simulink model "acf_rl_native"  (R2026b)
settings: Solver=ode4  StopTime=inf  FixedStep=3.3333333333333333e-06
InitFcn:
  | acf_select_actuator(bdroot);
model workspace (MAT data in the model file):
  acfControlVersion = 'force-observer-v1'
  acfImplementation = 'simple'
  acfLayoutVersion = 1
  p : object (value not decoded)
  pCompliant : object (value not decoded)
  pNearContact : object (value not decoded)
  pNoSprings : object (value not decoded)
  pRecommended : object (value not decoded)
symbols that are objects in the model workspace (value not decoded): p
undefined symbols (not defined in the file or in its folder): DiscIntNeverNeededParam
libraries: sl_discontinuities x1
(part 2 of 3)

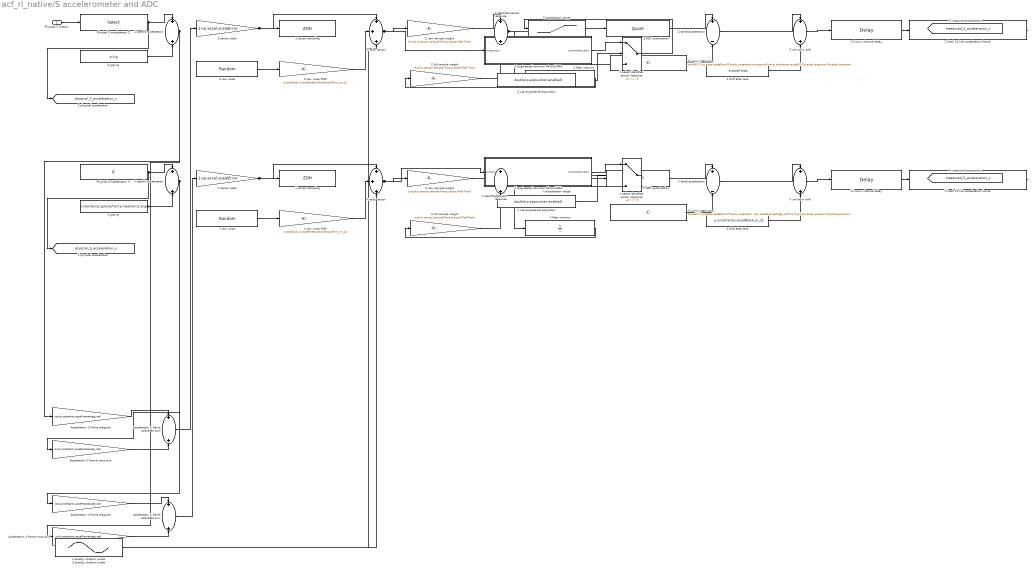
== system acf_rl_native/S accelerometer and ADC ==
  Physical S motion : Inport
  Acceleration X frame calibrated sum : Sum
  Acceleration X frame cross axis : Gain  Gain=-sin(p.uncertainty.accelFrameAngle_rad)
  Acceleration X frame diagonal : Gain  Gain=cos(p.uncertainty.accelFrameAngle_rad)
  Acceleration Z frame calibrated sum : Sum
  Acceleration Z frame cross axis : Gain  Gain=sin(p.uncertainty.accelFrameAngle_rad)
  Acceleration Z frame diagonal : Gain  Gain=cos(p.uncertainty.accelFrameAngle_rad)
  Physical S acceleration X : Constant  Value=0
  Physical S acceleration Z : Selector  InputPortWidth=3  IndexOptions=Index vector (dialog)  Indices=3  OutputSizes=1
  X ADC quantization : Quantizer  QuantizationInterval=1e-15
  X acceleration range : Saturate  UpperLimit=inf  LowerLimit=-inf
  X analog vibration probe : Sin  Amplitude=p.adcStudy.accelerationXAnalogToneAmplitude_m_s2  Frequency=2*pi*p.adcStudy.analogToneFrequency_Hz  Phase=p.adcStudy.analogTonePhase_rad  SampleTime=0
  X drift after tare : Constant  Value=p.uncertainty.accelBiasX_m_s2
  X engineered common AA and EMA : Subsystem
  X filter memory : UnitDelay  InitialCondition=(1+p.accel.scaleError)*(cos(p.uncertainty.accelFrameAngle_rad)*(p.mechanics.gravity*sin(p.mechanics.angle))-sin(p.uncertainty.accelFrameAngle_rad)*(p.d.g))  SampleTime=p.sensor.sampleTime
  X fresh 10 kHz acceleration frame : ZeroOrderHold  SampleTime=p.force.sampleTime
  X gravity : Constant  Value=p.mechanics.gravity*sin(p.mechanics.angle)
  X identified sensor response : Sum
  X known channel delay : TransportDelay  DelayTime=p.adcStudy.d.channels.acceleration.pipelineDelay_s  InitialOutput=p.uncertainty.accelBiasX_m_s2
  X known static tare : Constant  Value=round((((1+p.accel.scaleError)*(cos(p.uncertainty.accelFrameAngle_rad)*(p.mechanics.gravity*sin(p.mechanics.angle))-sin(p.uncertainty.accelFrameAngle_rad)*(p.d.g))))/p.accel.quantum)*p.accel.quantum
  X new sample weight : Gain  Gain=1-exp(-p.sensor.sampleTime/p.accel.filterTime)
  X noisy sensor : Sum  Inputs=+++
  X old sample weight : Gain  Gain=exp(-p.sensor.sampleTime/p.accel.filterTime)
  X raw noise : RandomNumber  Seed=p.sensor.seed+336  SampleTime=p.sensor.sampleTime
  X raw noise RMS : Gain  Gain=p.adcStudy.d.accelerationNoiseInputRms_m_s2
  X select identified sensor response : Switch  Threshold=.5  SaturateOnIntegerOverflow=off  InputSameDT=off
  X sensor sampling : ZeroOrderHold  SampleTime=p.sensor.sampleTime
  X sensor scale : Gain  Gain=1+p.accel.scaleError
  X specific acceleration : Sum
  X tared acceleration : Sum  Inputs=+-
  X unknown drift : Sum
  X use engineered acquisition : Constant  Value=double(p.acquisition.enabled)
  Z ADC quantization : Quantizer  QuantizationInterval=1e-15
  Z acceleration range : Saturate  UpperLimit=inf  LowerLimit=-inf
  Z analog vibration probe : Sin  Amplitude=p.adcStudy.accelerationZAnalogToneAmplitude_m_s2  Frequency=2*pi*p.adcStudy.analogToneFrequency_Hz  Phase=p.adcStudy.analogTonePhase_rad  SampleTime=0
  Z drift after tare : Constant  Value=p.accel.bias
  Z engineered common AA and EMA : Subsystem
  Z filter memory : UnitDelay  InitialCondition=(1+p.accel.scaleError)*(cos(p.uncertainty.accelFrameAngle_rad)*(p.d.g)+sin(p.uncertainty.accelFrameAngle_rad)*(p.mechanics.gravity*sin(p.mechanics.angle)))  SampleTime=p.sensor.sampleTime
  Z fresh 10 kHz acceleration frame : ZeroOrderHold  SampleTime=p.force.sampleTime
  Z gravity : Constant  Value=p.d.g
  Z identified sensor response : Sum
  Z known channel delay : TransportDelay  DelayTime=p.adcStudy.d.channels.acceleration.pipelineDelay_s  InitialOutput=p.accel.bias
  Z known static tare : Constant  Value=round((((1+p.accel.scaleError)*(cos(p.uncertainty.accelFrameAngle_rad)*(p.d.g)+sin(p.uncertainty.accelFrameAngle_rad)*(p.mechanics.gravity*sin(p.mechanics.angle)))))/p.accel.quantum)*p.accel.quantum
  Z new sample weight : Gain  Gain=1-exp(-p.sensor.sampleTime/p.accel.filterTime)
  Z noisy sensor : Sum  Inputs=+++
  Z old sample weight : Gain  Gain=exp(-p.sensor.sampleTime/p.accel.filterTime)
  Z raw noise : RandomNumber  Seed=p.sensor.seed+239  SampleTime=p.sensor.sampleTime
  Z raw noise RMS : Gain  Gain=p.adcStudy.d.accelerationNoiseInputRms_m_s2
  Z select identified sensor response : Switch  Threshold=.5  SaturateOnIntegerOverflow=off  InputSameDT=off
  Z sensor sampling : ZeroOrderHold  SampleTime=p.sensor.sampleTime
  Z sensor scale : Gain  Gain=1+p.accel.scaleError
  Z specific acceleration : Sum
  Z tared acceleration : Sum  Inputs=+-
  Z unknown drift : Sum
  Z use engineered acquisition : Constant  Value=double(p.acquisition.enabled)
  tag scope: measured_S_acceleration_x=global, measured_S_acceleration_z=global, physical_S_acceleration_x=global, physical_S_acceleration_z=global
  wires:
  Physical S motion/1 -> Physical S acceleration Z/1
  Physical S acceleration Z/1 -> [physical_S_acceleration_z], Z specific acceleration/1
  Z gravity/1 -> Z specific acceleration/2
  Z sensor scale/1 -> Z sensor sampling/1, Z noisy sensor/1
  Z raw noise/1 -> Z raw noise RMS/1
  Z raw noise RMS/1 -> Z noisy sensor/2
  Z noisy sensor/1 -> Z new sample weight/1, Z engineered common AA and EMA/1(analog input)
  Z new sample weight/1 -> Z identified sensor response/1
  Z identified sensor response/1 -> Z filter memory/1, Z select identified sensor response/3
  Z filter memory/1 -> Z old sample weight/1
  Z old sample weight/1 -> Z identified sensor response/2
  Z acceleration range/1 -> Z ADC quantization/1
  Z ADC quantization/1 -> Z tared acceleration/1
  Z known static tare/1 -> Z tared acceleration/2
  Z tared acceleration/1 -> Z unknown drift/1
  Z drift after tare/1 -> Z unknown drift/2
  Physical S acceleration X/1 -> [physical_S_acceleration_x], X specific acceleration/1
  X gravity/1 -> X specific acceleration/2
  X specific acceleration/1 -> Acceleration Z frame cross axis/1, Acceleration X frame diagonal/1
  X sensor scale/1 -> X sensor sampling/1, X noisy sensor/1
  X raw noise/1 -> X raw noise RMS/1
  X raw noise RMS/1 -> X noisy sensor/2
  X noisy sensor/1 -> X new sample weight/1, X engineered common AA and EMA/1(analog input)
  X new sample weight/1 -> X identified sensor response/1
  X identified sensor response/1 -> X filter memory/1, X select identified sensor response/3
  X filter memory/1 -> X old sample weight/1
  X old sample weight/1 -> X identified sensor response/2
  X acceleration range/1 -> X ADC quantization/1
  X ADC quantization/1 -> X tared acceleration/1
  X known static tare/1 -> X tared acceleration/2
  X tared acceleration/1 -> X unknown drift/1
  X drift after tare/1 -> X unknown drift/2
  Z use engineered acquisition/1 -> Z select identified sensor response/2
  Z select identified sensor response/1 -> Z acceleration range/1
  Z fresh 10 kHz acceleration frame/1 -> [measured_S_acceleration_z]
  X use engineered acquisition/1 -> X select identified sensor response/2
  X select identified sensor response/1 -> X acceleration range/1
  X fresh 10 kHz acceleration frame/1 -> [measured_S_acceleration_x]
  Z specific acceleration/1 -> Acceleration Z frame diagonal/1, Acceleration X frame cross axis/1
  Acceleration Z frame diagonal/1 -> Acceleration Z frame calibrated sum/1
  Acceleration Z frame cross axis/1 -> Acceleration Z frame calibrated sum/2
  Acceleration Z frame calibrated sum/1 -> Z sensor scale/1
  Acceleration X frame diagonal/1 -> Acceleration X frame calibrated sum/1
  Acceleration X frame cross axis/1 -> Acceleration X frame calibrated sum/2
  Acceleration X frame calibrated sum/1 -> X sensor scale/1
  Z analog vibration probe/1 -> Z noisy sensor/3
  Z engineered common AA and EMA/1(conditioned output) -> Z select identified sensor response/1
  Z unknown drift/1 -> Z known channel delay/1
  Z known channel delay/1 -> Z fresh 10 kHz acceleration frame/1
  X analog vibration probe/1 -> X noisy sensor/3
  X engineered common AA and EMA/1(conditioned output) -> X select identified sensor response/1
  X unknown drift/1 -> X known channel delay/1
  X known channel delay/1 -> X fresh 10 kHz acceleration frame/1

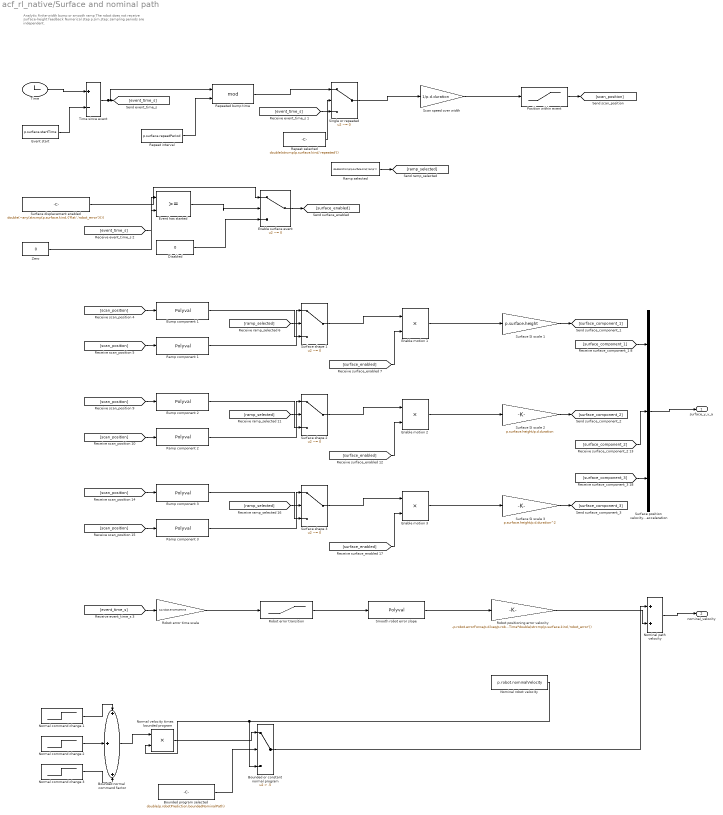
== system acf_rl_native/Surface and nominal path ==
  note: Analytic finite-width bump or smooth ramp
      | The robot does not receive surface-height feedback
      | Numerical step p.sim.step; sampling periods are independent.
  Bounded normal command factor : Sum  Inputs=+++
  Bounded or constant normal program : Switch  Criteria=u2 > Threshold  Threshold=.5  SaturateOnIntegerOverflow=off  InputSameDT=off
  Bounded program selected : Constant  Value=double(p.robotPrediction.boundedNominalPath)
  Bump component 1 : Polyval  Coefs=[-64 192 -192 64 0 0 0]
  Bump component 2 : Polyval  Coefs=[-384 960 -768 192 0 0]
  Bump component 3 : Polyval  Coefs=[-1920 3840 -2304 384 0]
  Disabled : Constant  Value=0
  Enable motion 1 : Product
  Enable motion 2 : Product
  Enable motion 3 : Product
  Enable surface event : Switch  Criteria=u2 ~= 0  SaturateOnIntegerOverflow=off  InputSameDT=off
  Event has started : RelationalOperator  OutDataTypeStr=boolean  RndMeth=Simplest  InputSameDT=off
  Event start : Constant  Value=p.surface.startTime
  Nominal path velocity : Sum
  Nominal robot velocity : Constant  Value=p.robot.nominalVelocity
  Normal command change 1 : Step  SampleTime=p.robot.sampleTime
  Normal command change 2 : Step  Time=2  FinalValue=-2  SampleTime=p.robot.sampleTime
  Normal command change 3 : Step  Time=3  SampleTime=p.robot.sampleTime
  Normal velocity times bounded program : Product
  Position within event : Saturate  UpperLimit=1  LowerLimit=0
  Ramp component 1 : Polyval  Coefs=[6 -15 10 0 0 0]
  Ramp component 2 : Polyval  Coefs=[30 -60 30 0 0]
  Ramp component 3 : Polyval  Coefs=[120 -180 60 0]
  Ramp selected : Constant  Value=double(strcmp(p.surface.kind,'ramp'))
  Repeat interval : Constant  Value=p.surface.repeatPeriod
  Repeat selected : Constant  Value=double(strcmp(p.surface.kind,'repeated'))
  Repeated bump time : Math  Operator=mod
  Robot error time scale : Gain  Gain=1/p.robot.errorRiseTime
  Robot error transition : Saturate  UpperLimit=1  LowerLimit=0
  Robot positioning error velocity : Gain  Gain=-p.robot.errorForce/p.d.keq/p.robot.errorRiseTime*double(strcmp(p.surface.kind,'robot_error'))
  Scan speed over width : Gain  Gain=1/p.d.duration
  Single or repeated : Switch  Criteria=u2 ~= 0  SaturateOnIntegerOverflow=off  InputSameDT=off
  Smooth robot error slope : Polyval  Coefs=[30 -60 30 0 0]
  Surface SI scale 1 : Gain  Gain=p.surface.height
  Surface SI scale 2 : Gain  Gain=p.surface.height/p.d.duration
  Surface SI scale 3 : Gain  Gain=p.surface.height/p.d.duration^2
  Surface displacement enabled : Constant  Value=double(~any(strcmp(p.surface.kind,{'flat','robot_error'})))
  Surface position velocity acceleration : Mux  Inputs=3
  Surface shape 1 : Switch  Criteria=u2 ~= 0  SaturateOnIntegerOverflow=off  InputSameDT=off
  Surface shape 2 : Switch  Criteria=u2 ~= 0  SaturateOnIntegerOverflow=off  InputSameDT=off
  Surface shape 3 : Switch  Criteria=u2 ~= 0  SaturateOnIntegerOverflow=off  InputSameDT=off
  Time : Clock
  Time since event : Sum  Inputs=+-
  Zero : Constant  Value=0
  surface_y_v_a : Outport
  nominal_velocity : Outport  Port=2
  wires:
  [scan_position] -> Bump component 1/1
  [scan_position] -> Bump component 2/1
  [scan_position] -> Bump component 3/1
  Surface shape 1/1 -> Enable motion 1/1
  [surface_enabled] -> Enable motion 1/2
  Surface shape 2/1 -> Enable motion 2/1
  [surface_enabled] -> Enable motion 2/2
  Surface shape 3/1 -> Enable motion 3/1
  [surface_enabled] -> Enable motion 3/2
  Surface displacement enabled/1 -> Enable surface event/1
  Event has started/1 -> Enable surface event/2
  Disabled/1 -> Enable surface event/3
  [event_time_s] -> Event has started/1
  Zero/1 -> Event has started/2
  Robot positioning error velocity/1 -> Nominal path velocity/2
  Scan speed over width/1 -> Position within event/1
  [scan_position] -> Ramp component 1/1
  [scan_position] -> Ramp component 2/1
  [scan_position] -> Ramp component 3/1
  Time since event/1 -> Repeated bump time/1, [event_time_s]
  Repeat interval/1 -> Repeated bump time/2
  [event_time_s] -> Robot error time scale/1
  Robot error time scale/1 -> Robot error transition/1
  Smooth robot error slope/1 -> Robot positioning error velocity/1
  Single or repeated/1 -> Scan speed over width/1
  Ramp selected/1 -> [ramp_selected]
  Position within event/1 -> [scan_position]
  Surface SI scale 1/1 -> [surface_component_1]
  Surface SI scale 2/1 -> [surface_component_2]
  Surface SI scale 3/1 -> [surface_component_3]
  Enable surface event/1 -> [surface_enabled]
  Repeated bump time/1 -> Single or repeated/1
  Repeat selected/1 -> Single or repeated/2
  [event_time_s] -> Single or repeated/3
  Robot error transition/1 -> Smooth robot error slope/1
  Enable motion 1/1 -> Surface SI scale 1/1
  Enable motion 2/1 -> Surface SI scale 2/1
  Enable motion 3/1 -> Surface SI scale 3/1
  [surface_component_1] -> Surface position velocity acceleration/1
  [surface_component_2] -> Surface position velocity acceleration/2
  [surface_component_3] -> Surface position velocity acceleration/3
  Ramp component 1/1 -> Surface shape 1/1
  [ramp_selected] -> Surface shape 1/2
  Bump component 1/1 -> Surface shape 1/3
  Ramp component 2/1 -> Surface shape 2/1
  [ramp_selected] -> Surface shape 2/2
  Bump component 2/1 -> Surface shape 2/3
  Ramp component 3/1 -> Surface shape 3/1
  [ramp_selected] -> Surface shape 3/2
  Bump component 3/1 -> Surface shape 3/3
  Time/1 -> Time since event/1
  Event start/1 -> Time since event/2
  Surface position velocity acceleration/1 -> surface_y_v_a/1
  Nominal path velocity/1 -> nominal_velocity/1
  Normal command change 1/1 -> Bounded normal command factor/1
  Normal command change 2/1 -> Bounded normal command factor/2
  Normal command change 3/1 -> Bounded normal command factor/3
  Bounded normal command factor/1 -> Normal velocity times bounded program/1
  Nominal robot velocity/1 -> Normal velocity times bounded program/2, Bounded or constant normal program/3
  Normal velocity times bounded program/1 -> Bounded or constant normal program/1
  Bounded program selected/1 -> Bounded or constant normal program/2
  Bounded or constant normal program/1 -> Nominal path velocity/1

== system acf_rl_native/Surface contact force ==
  Axial reaction : Inport
  Physical surface velocity : Inport  Port=2
  Axial reaction factor : Sum  Inputs=+-
  Friction times slope : Gain  Gain=p.contact.mu
  Lateral reaction : Product  Inputs=**/
  Lateral sign : Gain  Gain=-1
  Normal reaction : Product  Inputs=**/
  Normalizer : Math  Operator=sqrt
  Slope plus friction : Bias  Bias=p.contact.mu  SaturateOnIntegerOverflow=off
  Squared slope : Math  Operator=square
  Squared slope plus one : Bias  Bias=1  SaturateOnIntegerOverflow=off
  Surface slope : Gain  Gain=1/p.surface.scanSpeed
  Unity : Constant
  Velocity component : Selector  InputPortWidth=3  IndexOptions=Index vector (dialog)  Indices=2  OutputSizes=1
  tag scope: actual_contact_slope=global, lateral_contact_N=global, normal_contact_N=global
  wires:
  Physical surface velocity/1 -> Velocity component/1
  Velocity component/1 -> Surface slope/1
  Surface slope/1 -> Squared slope/1, Friction times slope/1, Slope plus friction/1, [actual_contact_slope]
  Squared slope/1 -> Squared slope plus one/1
  Squared slope plus one/1 -> Normalizer/1
  Unity/1 -> Axial reaction factor/1
  Friction times slope/1 -> Axial reaction factor/2
  Axial reaction/1 -> Normal reaction/1
  Normalizer/1 -> Normal reaction/2, Lateral reaction/3
  Axial reaction factor/1 -> Normal reaction/3
  Normal reaction/1 -> Lateral reaction/1, [normal_contact_N]
  Slope plus friction/1 -> Lateral reaction/2
  Lateral reaction/1 -> Lateral sign/1
  Lateral sign/1 -> [lateral_contact_N]

== system acf_rl_native/Actuator and RABS mechanics/Actuator ==
  Command : Inport
  Gap position velocity : Inport  Port=2
  Spring load : Inport  Port=3
  Ideal position : Subsystem  VariantControl=Ideal position
  Leadscrew : Subsystem  VariantControl=Leadscrew
  Voice coil : Subsystem  VariantControl=Voice coil
  Transmitted force : Outport
  Drive measurements : Outport  Port=2

== system acf_rl_native/Actuator and RABS mechanics/B to S spring and damper ==
  S position velocity : Inport
  B position velocity : Inport  Port=2
  Rigid reaction : Inport  Port=3
  Compliant or rigid link : VariantSource  VariantControlMode=label  LabelModeActiveChoice=Compliant  VariantControls={Compliant, Rigid}
  Damping : Gain  Gain=p.mechanics.c1
  Endpoint difference : Sum  Inputs=+-
  Preload : Constant  Value=p.d.q10
  Spring and damper force : Sum  Inputs=+++
  Spring displacement and relative velocity : Demux  Outputs=2
  Stiffness : Gain  Gain=p.mechanics.k1
  Spring force : Outport
  wires:
  Spring displacement and relative velocity/2 -> Damping/1
  S position velocity/1 -> Endpoint difference/1
  B position velocity/1 -> Endpoint difference/2
  Preload/1 -> Spring and damper force/1
  Stiffness/1 -> Spring and damper force/2
  Damping/1 -> Spring and damper force/3
  Endpoint difference/1 -> Spring displacement and relative velocity/1
  Spring displacement and relative velocity/1 -> Stiffness/1
  Spring and damper force/1 -> Compliant or rigid link/1
  Rigid reaction/1 -> Compliant or rigid link/2
  Compliant or rigid link/1 -> Spring force/1

== system acf_rl_native/Actuator and RABS mechanics/Mass A ==
  Actuator force : Inport
  Upper spring force : Inport  Port=2
  Gravity : Constant  Value=p.d.g
  Inverse mass : Gain  Gain=1/p.mechanics.mA
  Net applied force : Sum  Inputs=+-
  Newton acceleration : Sum  Inputs=+-
  Position : Integrator  InitialCondition=p.d.u0
  Position and velocity : Mux  Inputs=2
  Velocity : Integrator
  Position velocity : Outport
  Acceleration : Outport  Port=2
  wires:
  Net applied force/1 -> Inverse mass/1
  Actuator force/1 -> Net applied force/1
  Upper spring force/1 -> Net applied force/2
  Inverse mass/1 -> Newton acceleration/1
  Gravity/1 -> Newton acceleration/2
  Velocity/1 -> Position/1, [velocity_m_s]
  Position/1 -> Position and velocity/1
  [velocity_m_s] -> Position and velocity/2
  Newton acceleration/1 -> Velocity/1, Acceleration/1
  Position and velocity/1 -> Position velocity/1

== system acf_rl_native/Actuator and RABS mechanics/Mass B ==
  Lower spring force : Inport
  Actuator force : Inport  Port=2
  Gravity : Constant  Value=p.d.g
  Inverse mass : Gain  Gain=1/p.mechanics.mB
  Net applied force : Sum  Inputs=+-
  Newton acceleration : Sum  Inputs=+-
  Position : Integrator
  Position and velocity : Mux  Inputs=2
  Velocity : Integrator
  Position velocity : Outport
  Acceleration : Outport  Port=2
  wires:
  Net applied force/1 -> Inverse mass/1
  Lower spring force/1 -> Net applied force/1
  Actuator force/1 -> Net applied force/2
  Inverse mass/1 -> Newton acceleration/1
  Gravity/1 -> Newton acceleration/2
  Velocity/1 -> Position/1, [velocity_m_s]
  Position/1 -> Position and velocity/1
  [velocity_m_s] -> Position and velocity/2
  Newton acceleration/1 -> Velocity/1, Acceleration/1
  Position and velocity/1 -> Position velocity/1

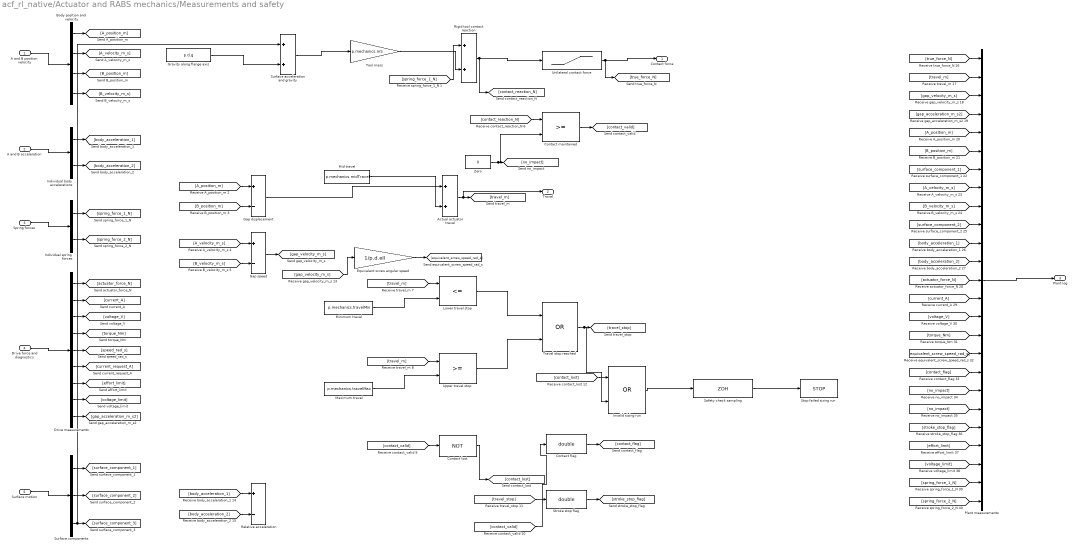
== system acf_rl_native/Actuator and RABS mechanics/Measurements and safety ==
  A and B position velocity : Inport
  A and B acceleration : Inport  Port=2
  Spring forces : Inport  Port=3
  Drive force and diagnostics : Inport  Port=4
  Surface motion : Inport  Port=5
  Actual actuator travel : Sum
  Body position and velocity : Demux
  Contact flag : DataTypeConversion  OutDataTypeStr=double  SaturateOnIntegerOverflow=off  RndMeth=Floor
  Contact lost : Logic  Operator=NOT  AllPortsSameDT=off  OutDataTypeStr=boolean
  Contact maintained : RelationalOperator  OutDataTypeStr=boolean  RndMeth=Simplest  InputSameDT=off
  Drive measurements : Demux  Outputs=9
  Equivalent screw angular speed : Gain  Gain=1/p.d.ell
  Gap displacement : Sum  Inputs=+-
  Gap speed : Sum  Inputs=+-
  Gravity along flange axis : Constant  Value=p.d.g
  Individual body accelerations : Demux  Outputs=2
  Individual spring forces : Demux  Outputs=2
  Invalid sizing run : Logic  Operator=OR  AllPortsSameDT=off  OutDataTypeStr=boolean
  Lower travel stop : RelationalOperator  Operator=<=  OutDataTypeStr=boolean  RndMeth=Simplest  InputSameDT=off
  Maximum travel : Constant  Value=p.mechanics.travelMax
  Mid travel : Constant  Value=p.mechanics.midTravel
  Minimum travel : Constant  Value=p.mechanics.travelMin
  Plant measurements : Mux  Inputs=25
  Relative acceleration : Sum  Inputs=+-
  Rigid tool contact reaction : Sum
  Safety check sampling : ZeroOrderHold  SampleTime=p.sim.step
  Stop failed sizing run : Stop
  Stroke stop flag : DataTypeConversion  OutDataTypeStr=double  SaturateOnIntegerOverflow=off  RndMeth=Floor
  Surface acceleration and gravity : Sum
  Surface components : Demux  Outputs=3
  Tool mass : Gain  Gain=p.mechanics.mS
  Travel stop reached : Logic  Operator=OR  AllPortsSameDT=off  OutDataTypeStr=boolean
  Unilateral contact force : Saturate  UpperLimit=inf  LowerLimit=0
  Upper travel stop : RelationalOperator  OutDataTypeStr=boolean  RndMeth=Simplest  InputSameDT=off
  Zero : Constant  Value=0
  Contact force : Outport
  Travel : Outport  Port=2
  Plant log : Outport  Port=3
  wires:
  Gap displacement/1 -> Actual actuator travel/1
  Mid travel/1 -> Actual actuator travel/2
  A and B position velocity/1 -> Body position and velocity/1
  [contact_valid] -> Contact flag/1
  [contact_valid] -> Contact lost/1
  [contact_reaction_N] -> Contact maintained/1
  Zero/1 -> Contact maintained/2, [no_impact]
  Drive force and diagnostics/1 -> Drive measurements/1
  [gap_velocity_m_s] -> Equivalent screw angular speed/1
  [A_position_m] -> Gap displacement/1
  [B_position_m] -> Gap displacement/2
  [A_velocity_m_s] -> Gap speed/1
  [B_velocity_m_s] -> Gap speed/2
  A and B acceleration/1 -> Individual body accelerations/1
  Spring forces/1 -> Individual spring forces/1
  [contact_lost] -> Invalid sizing run/1
  Travel stop reached/1 -> Invalid sizing run/2, [travel_stop]
  [travel_m] -> Lower travel stop/1
  Minimum travel/1 -> Lower travel stop/2
  [true_force_N] -> Plant measurements/1
  [travel_m] -> Plant measurements/2
  [gap_velocity_m_s] -> Plant measurements/3
  [gap_acceleration_m_s2] -> Plant measurements/4
  [A_position_m] -> Plant measurements/5
  [B_position_m] -> Plant measurements/6
  [surface_component_1] -> Plant measurements/7
  [A_velocity_m_s] -> Plant measurements/8
  [B_velocity_m_s] -> Plant measurements/9
  [surface_component_2] -> Plant measurements/10
  [body_acceleration_1] -> Plant measurements/11
  [body_acceleration_2] -> Plant measurements/12
  [actuator_force_N] -> Plant measurements/13
  [current_A] -> Plant measurements/14
  [voltage_V] -> Plant measurements/15
  [torque_Nm] -> Plant measurements/16
  [equivalent_screw_speed_rad_s] -> Plant measurements/17
  [contact_flag] -> Plant measurements/18
  [no_impact] -> Plant measurements/19
  [no_impact] -> Plant measurements/20
  [stroke_stop_flag] -> Plant measurements/21
  [effort_limit] -> Plant measurements/22
  [voltage_limit] -> Plant measurements/23
  [spring_force_1_N] -> Plant measurements/24
  [spring_force_2_N] -> Plant measurements/25
  [body_acceleration_1] -> Relative acceleration/1
  [body_acceleration_2] -> Relative acceleration/2
  [spring_force_1_N] -> Rigid tool contact reaction/1
  Tool mass/1 -> Rigid tool contact reaction/2
  Invalid sizing run/1 -> Safety check sampling/1
  Body position and velocity/1 -> [A_position_m]
  Body position and velocity/2 -> [A_velocity_m_s]
  Body position and velocity/3 -> [B_position_m]
  Body position and velocity/4 -> [B_velocity_m_s]
  Drive measurements/1 -> [actuator_force_N]
  Individual body accelerations/1 -> [body_acceleration_1]
  Individual body accelerations/2 -> [body_acceleration_2]
  Contact flag/1 -> [contact_flag]
  Contact lost/1 -> [contact_lost]
  Rigid tool contact reaction/1 -> [contact_reaction_N], Unilateral contact force/1
  Contact maintained/1 -> [contact_valid]
  Drive measurements/2 -> [current_A]
  Drive measurements/6 -> [current_request_A]
  Drive measurements/7 -> [effort_limit]
  Equivalent screw angular speed/1 -> [equivalent_screw_speed_rad_s]
  Drive measurements/9 -> [gap_acceleration_m_s2]
  Gap speed/1 -> [gap_velocity_m_s]
  Drive measurements/5 -> [speed_rad_s]
  Individual spring forces/1 -> [spring_force_1_N]
  Individual spring forces/2 -> [spring_force_2_N]
  Stroke stop flag/1 -> [stroke_stop_flag]
  Surface components/1 -> [surface_component_1]
  Surface components/2 -> [surface_component_2]
  Surface components/3 -> [surface_component_3], Surface acceleration and gravity/1
  Drive measurements/4 -> [torque_Nm]
  Actual actuator travel/1 -> [travel_m], Travel/1
  Unilateral contact force/1 -> [true_force_N], Contact force/1
  Drive measurements/3 -> [voltage_V]
  Drive measurements/8 -> [voltage_limit]
  Safety check sampling/1 -> Stop failed sizing run/1
  [travel_stop] -> Stroke stop flag/1
  Gravity along flange axis/1 -> Surface acceleration and gravity/2
  Surface motion/1 -> Surface components/1
  Surface acceleration and gravity/1 -> Tool mass/1
  Lower travel stop/1 -> Travel stop reached/1
  Upper travel stop/1 -> Travel stop reached/2
  [travel_m] -> Upper travel stop/1
  Maximum travel/1 -> Upper travel stop/2
  Plant measurements/1 -> Plant log/1

== system acf_rl_native/Actuator and RABS mechanics/R to A spring and damper ==
  A position velocity : Inport
  R position velocity : Inport  Port=2
  Rigid reaction : Inport  Port=3
  Compliant or rigid link : VariantSource  VariantControlMode=label  LabelModeActiveChoice=Rigid  VariantControls={Compliant, Rigid}
  Damping : Gain  Gain=p.mechanics.c2
  Endpoint difference : Sum  Inputs=+-
  Preload : Constant  Value=p.d.q20
  Spring and damper force : Sum  Inputs=+++
  Spring displacement and relative velocity : Demux  Outputs=2
  Stiffness : Gain  Gain=p.mechanics.k2
  Spring force : Outport
  wires:
  Spring displacement and relative velocity/2 -> Damping/1
  A position velocity/1 -> Endpoint difference/1
  R position velocity/1 -> Endpoint difference/2
  Preload/1 -> Spring and damper force/1
  Stiffness/1 -> Spring and damper force/2
  Damping/1 -> Spring and damper force/3
  Endpoint difference/1 -> Spring displacement and relative velocity/1
  Spring displacement and relative velocity/1 -> Stiffness/1
  Spring and damper force/1 -> Compliant or rigid link/1
  Rigid reaction/1 -> Compliant or rigid link/2
  Compliant or rigid link/1 -> Spring force/1

== system acf_rl_native/Contact force measurement/Contact force reconstruction ==
  raw_cell_error_N : Inport
  Cell error to deviation : Gain  Gain=-1
  Compensated axial reaction : Sum
  Compensated lateral reaction : Sum
  Downstream X inertia : Gain  Gain=p.sensor.distalMass_model_kg
  Downstream Z inertia : Gain  Gain=p.sensor.distalMass_model_kg
  Tared axial cell force : Bias  Bias=p.force.reference  SaturateOnIntegerOverflow=off
  axial_contact_N : Outport
  lateral_contact_N : Outport  Port=2
  tag scope: inertial_axial_contact_N=global, inertial_lateral_contact_N=global
  wires:
  Compensated axial reaction/1 -> axial_contact_N/1, [inertial_axial_contact_N]
  Tared axial cell force/1 -> Compensated axial reaction/1
  Downstream Z inertia/1 -> Compensated axial reaction/2
  Compensated lateral reaction/1 -> lateral_contact_N/1, [inertial_lateral_contact_N]
  Cell error to deviation/1 -> Tared axial cell force/1
  [measured_S_acceleration_z] -> Downstream Z inertia/1
  [measured_lateral_contact_N] -> Compensated lateral reaction/1
  Downstream X inertia/1 -> Compensated lateral reaction/2
  raw_cell_error_N/1 -> Cell error to deviation/1
  [measured_S_acceleration_x] -> Downstream X inertia/1

== system acf_rl_native/Contact force measurement/Head motion estimator ==
  measured_head_position_m : Inport
  Causal motion measurements : Mux  Inputs=3
  Estimated head travel : Bias  Bias=p.mechanics.midTravel+p.d.u0  SaturateOnIntegerOverflow=off
  Fresh 10 kHz position frame : ZeroOrderHold  SampleTime=p.force.sampleTime
  Fresh 10 kHz robot acceleration frame : ZeroOrderHold  SampleTime=p.force.sampleTime
  Fresh 10 kHz robot velocity frame : ZeroOrderHold  SampleTime=p.force.sampleTime
  Head gap and velocity observer : DiscreteStateSpace  A=p.d.toolMotionObserver.A  B=p.d.toolMotionObserver.B  C=p.d.toolMotionObserver.C  D=p.d.toolMotionObserver.D  InitialCondition=zeros(2,1)  SampleTime=p.force.sampleTime
  Head gap coordinate sign : Gain  Gain=-1
  Head gap displacement : Selector  InputPortWidth=2  IndexOptions=Index vector (dialog)  Indices=1  OutputSizes=1
  Head gap velocity : Selector  InputPortWidth=2  IndexOptions=Index vector (dialog)  Indices=2  OutputSizes=1
  Measured head coordinate deviation : Bias  Bias=p.d.positionMeasurementBias  SaturateOnIntegerOverflow=off
  Position ADC delivery pipeline : TransportDelay  DelayTime=p.adcStudy.d.channels.position.pipelineDelay_s
  Position acquisition frame : Switch  Threshold=.5  SaturateOnIntegerOverflow=off  InputSameDT=off
  Position common AA and EMA : Subsystem
  Position frame matching : DiscreteStateSpace  A=exp(-p.sensor.sampleTime/p.sensor.filterTime)  B=1-exp(-p.sensor.sampleTime/p.sensor.filterTime)  C=exp(-p.sensor.sampleTime/p.sensor.filterTime)  D=1-exp(-p.sensor.sampleTime/p.sensor.filterTime)  SampleTime=p.sensor.sampleTime
  Position use engineered acquisition : Constant  Value=double(p.acquisition.enabled)
  Robot acceleration acquisition frame : Switch  Threshold=.5  SaturateOnIntegerOverflow=off  InputSameDT=off
  Robot acceleration common AA and EMA : Subsystem
  Robot acceleration frame matching : DiscreteStateSpace  A=exp(-p.sensor.sampleTime/p.sensor.filterTime)  B=1-exp(-p.sensor.sampleTime/p.sensor.filterTime)  C=exp(-p.sensor.sampleTime/p.sensor.filterTime)  D=1-exp(-p.sensor.sampleTime/p.sensor.filterTime)  SampleTime=p.sensor.sampleTime
  Robot acceleration frame matching delay : TransportDelay  DelayTime=p.adcStudy.d.channels.frame.pipelineDelay_s
  Robot acceleration use engineered acquisition : Constant  Value=double(p.acquisition.enabled)
  Robot velocity acquisition frame : Switch  Threshold=.5  SaturateOnIntegerOverflow=off  InputSameDT=off
  Robot velocity common AA and EMA : Subsystem
  Robot velocity frame matching : DiscreteStateSpace  A=exp(-p.sensor.sampleTime/p.sensor.filterTime)  B=1-exp(-p.sensor.sampleTime/p.sensor.filterTime)  C=exp(-p.sensor.sampleTime/p.sensor.filterTime)  D=1-exp(-p.sensor.sampleTime/p.sensor.filterTime)  SampleTime=p.sensor.sampleTime
  Robot velocity frame matching delay : TransportDelay  DelayTime=p.adcStudy.d.channels.frame.pipelineDelay_s
  Robot velocity use engineered acquisition : Constant  Value=double(p.acquisition.enabled)
  head_gap_velocity_m_s : Outport
  estimated_head_travel_m : Outport  Port=2
  tag scope: inertial_head_motion_states=global, inertial_robot_acceleration_aligned=global, inertial_robot_velocity_aligned=global, rl_aligned_relative_position=global
  wires:
  Estimated head travel/1 -> estimated_head_travel_m/1
  measured_head_position_m/1 -> Measured head coordinate deviation/1
  Head gap velocity/1 -> head_gap_velocity_m_s/1
  [command_based_robot_velocity] -> Robot velocity frame matching/1, Robot velocity common AA and EMA/1(analog input)
  Measured head coordinate deviation/1 -> Head gap coordinate sign/1
  [command_based_robot_acceleration] -> Robot acceleration frame matching/1, Robot acceleration common AA and EMA/1(analog input)
  Head gap coordinate sign/1 -> Position frame matching/1, Position common AA and EMA/1(analog input)
  Causal motion measurements/1 -> Head gap and velocity observer/1
  Head gap displacement/1 -> Estimated head travel/1
  Head gap and velocity observer/1 -> Head gap displacement/1, Head gap velocity/1, [inertial_head_motion_states]
  [measured_S_acceleration_z] -> Causal motion measurements/3
  Position use engineered acquisition/1 -> Position acquisition frame/2
  Position frame matching/1 -> Position acquisition frame/3
  Fresh 10 kHz position frame/1 -> Causal motion measurements/1, [rl_aligned_relative_position]
  Robot acceleration use engineered acquisition/1 -> Robot acceleration acquisition frame/2
  Robot acceleration frame matching/1 -> Robot acceleration acquisition frame/3
  Fresh 10 kHz robot acceleration frame/1 -> [inertial_robot_acceleration_aligned], Causal motion measurements/2
  Robot velocity use engineered acquisition/1 -> Robot velocity acquisition frame/2
  Robot velocity frame matching/1 -> Robot velocity acquisition frame/3
  Fresh 10 kHz robot velocity frame/1 -> [inertial_robot_velocity_aligned]
  Position common AA and EMA/1(conditioned output) -> Position acquisition frame/1
  Robot velocity common AA and EMA/1(conditioned output) -> Robot velocity acquisition frame/1
  Robot acceleration common AA and EMA/1(conditioned output) -> Robot acceleration acquisition frame/1
  Robot velocity acquisition frame/1 -> Robot velocity frame matching delay/1
  Robot velocity frame matching delay/1 -> Fresh 10 kHz robot velocity frame/1
  Robot acceleration acquisition frame/1 -> Robot acceleration frame matching delay/1
  Robot acceleration frame matching delay/1 -> Fresh 10 kHz robot acceleration frame/1
  Position acquisition frame/1 -> Position ADC delivery pipeline/1
  Position ADC delivery pipeline/1 -> Fresh 10 kHz position frame/1

== system acf_rl_native/Contact force measurement/Normal force projection ==
  Compensated axial force : Inport
  Compensated lateral force : Inport  Port=2
  Head gap velocity : Inport  Port=3
  Axial reference deviation : Bias  Bias=-p.force.reference  SaturateOnIntegerOverflow=off
  Causal surface direction : Gain  Gain=1/p.contact.commandedScanSpeed_m_s
  Estimated S velocity : Sum  Inputs=+-
  Lateral projection : Product  Inputs=**
  Measured drag audit vector : Mux  Inputs=3
  Measured drag geometry : Subsystem
  Measured drag geometry selected : Constant  Value=double(strcmp(p.contact.geometryMode,'measured_drag_ratio'))
  Measured drag native log : ToWorkspace  Commented=on  VariableName=measured_drag_log  SaveFormat=Timeseries  SampleTime=-1
  Measured drag native sample 1 : ZeroOrderHold  SampleTime=p.sim.step
  Measured drag native sample 2 : ZeroOrderHold  SampleTime=p.sim.step
  Measured drag native sample 3 : ZeroOrderHold  SampleTime=p.sim.step
  Measured normal force : Product  Inputs=*/
  Measured normal force deviation : Bias  Bias=-p.force.reference  SaturateOnIntegerOverflow=off
  Normal projection numerator : Sum  Inputs=+-
  Normal reference projection : Gain  Gain=p.force.reference
  Normalizer : Math  Operator=sqrt
  Requested axial force : Sum
  Select axial force geometry request : Switch  Threshold=.5  SaturateOnIntegerOverflow=off  InputSameDT=off
  Squared slope : Math  Operator=square
  Squared slope plus one : Bias  Bias=1  SaturateOnIntegerOverflow=off
  normal_force_deviation_N : Outport
  axial_reference_deviation_N : Outport  Port=2
  tag scope: estimated_contact_slope=global, estimated_normal_contact_N=global, requested_axial_contact_N=global
  wires:
  Axial reference deviation/1 -> axial_reference_deviation_N/1
  Measured normal force deviation/1 -> normal_force_deviation_N/1
  Head gap velocity/1 -> Estimated S velocity/2
  [inertial_robot_velocity_aligned] -> Estimated S velocity/1
  Squared slope/1 -> Squared slope plus one/1
  Compensated lateral force/1 -> Lateral projection/1, Measured drag geometry/2(reconstructed_Rx_N)
  Lateral projection/1 -> Normal projection numerator/2, Requested axial force/2
  Estimated S velocity/1 -> Causal surface direction/1
  Compensated axial force/1 -> Normal projection numerator/1, Measured drag geometry/1(reconstructed_Rz_N)
  Normal reference projection/1 -> Requested axial force/1
  Normal projection numerator/1 -> Measured normal force/1
  Normalizer/1 -> Measured normal force/2, Normal reference projection/1, Measured drag geometry/5(normalizer)
  Causal surface direction/1 -> Squared slope/1, [estimated_contact_slope], Lateral projection/2, Measured drag geometry/3(estimated_slope)
  Squared slope plus one/1 -> Normalizer/1
  Measured normal force/1 -> Measured normal force deviation/1, [estimated_normal_contact_N], Measured drag geometry/4(estimated_normal_N)
  Measured drag geometry/1(requested_Rz_N) -> Select axial force geometry request/1
  Measured drag geometry selected/1 -> Select axial force geometry request/2
  Requested axial force/1 -> Select axial force geometry request/3
  Select axial force geometry request/1 -> Axial reference deviation/1, [requested_axial_contact_N]
  Measured drag geometry/2(filtered_drag_ratio) -> Measured drag native sample 1/1
  Measured drag native sample 1/1 -> Measured drag audit vector/1
  Measured drag geometry/3(bounded_raw_drag_ratio) -> Measured drag native sample 2/1
  Measured drag native sample 2/1 -> Measured drag audit vector/2
  Measured drag geometry/4(drag_estimate_valid) -> Measured drag native sample 3/1
  Measured drag native sample 3/1 -> Measured drag audit vector/3
  Measured drag audit vector/1 -> Measured drag native log/1

== system acf_rl_native/Force controller/Coil PI and PID ==
  error_N : Inport
  measured_travel_m : Inport  Port=2
  Baseline or external current : Switch  Criteria=u2 > Threshold  Threshold=.5  SaturateOnIntegerOverflow=off  InputSameDT=off
  Current limits : Saturate  UpperLimit=p.coil.peakCurrent  LowerLimit=-p.coil.peakCurrent
  Current saturation error : Sum  Inputs=+-
  Flat holding current : Constant  Value=(p.force.reference-(p.uncertainty.massB_model_kg+p.sensor.distalMass_model_kg)*p.d.g)/p.uncertainty.forceConstant_model_N_A
  Integral anti windup : Gain  Gain=-p.force.antiWindupRate/p.inertial.forceKi
  Lower spring inverse feedforward : Subsystem
  Measured motion feedforward : Subsystem
  Normal force PI and PID : Subsystem
  Optional structural-mode current notch : DiscreteTransferFcn  Numerator=p.d.currentNotch.numerator  Denominator=p.d.currentNotch.denominator  InitialStates=p.d.currentNotch.initialStates  SampleTime=p.force.sampleTime
  PI PID and feedforward current : Sum  Inputs=++++++
  command : Outport
  estimated_travel_m : Outport  Port=2
  estimated_force_error_N : Outport  Port=3
  tag scope: rl_baseline_current=global, rl_equilibrium_current=global, rl_issued_current=global
  wires:
  measured_travel_m/1 -> estimated_travel_m/1
  Optional structural-mode current notch/1 -> Current limits/1, Current saturation error/2
  Integral anti windup/1 -> Normal force PI and PID/2(anti_windup)
  Current limits/1 -> command/1, Current saturation error/1, [rl_issued_current]
  PI PID and feedforward current/1 -> [rl_baseline_current], Baseline or external current/1
  Current saturation error/1 -> Integral anti windup/1
  error_N/1 -> estimated_force_error_N/1, Normal force PI and PID/1(error_N)
  Flat holding current/1 -> PI PID and feedforward current/1, [rl_equilibrium_current]
  Normal force PI and PID/1(feedback_current_A) -> PI PID and feedforward current/2
  Measured motion feedforward/1(acceleration_current_A) -> PI PID and feedforward current/3
  Measured motion feedforward/2(geometry_current_A) -> PI PID and feedforward current/4
  Measured motion feedforward/3(friction_current_A) -> PI PID and feedforward current/5
  Lower spring inverse feedforward/1(extra_current_A) -> PI PID and feedforward current/6
  [rl_baseline_mode] -> Baseline or external current/2
  [rl_external_current] -> Baseline or external current/3
  Baseline or external current/1 -> Optional structural-mode current notch/1

== system acf_rl_native/Force controller/Drive PI and PID ==
  note: Sampled PI + anti-windup
      | Coil: amperes; screw: rad/s; ideal: gap in metres
      | Numerical step p.sim.step; sampling periods are independent.
  note: PI / FILTERED PID
      | Kp, Ki, Kd and derivative-filter time are ordinary parameters.
      | Kd = 0 disables derivative action. Voice-coil strategy chooses this page or the observer.
  error_N : Inport
  measured_travel_m : Inport  Port=2
  Actuator command limits : Saturate  UpperLimit=p.d.commandMax  LowerLimit=p.d.commandMin
  Anti windup : Gain  Gain=p.force.antiWindupRate
  Derivative gain : Gain  Gain=p.d.forceKd*double(strcmp(p.coil.strategy,'pid'))
  Filtered force derivative : DiscreteTransferFcn  Numerator=(1-exp(-p.force.sampleTime/p.d.derivativeFilter))/p.force.sampleTime*[1 -1]  Denominator=[1 -exp(-p.force.sampleTime/p.d.derivativeFilter)]  SampleTime=p.force.sampleTime
  Force controller sampling : ZeroOrderHold  SampleTime=p.force.sampleTime
  Holding command : Constant  Value=p.d.forceFeedforward
  Integral action : DiscreteIntegrator  SampleTime=p.force.sampleTime  ICPrevOutput=DiscIntNeverNeededParam  ICPrevScaledInput=DiscIntNeverNeededParam
  Integral gain : Gain  Gain=p.d.forceKi
  Integral input : Sum
  PI plus holding command : Sum  Inputs=++++
  Proportional gain : Gain  Gain=p.d.forceKp
  Saturation error : Sum  Inputs=+-
  command : Outport
  estimated_travel_m : Outport  Port=2
  estimated_force_error_N : Outport  Port=3
  wires:
  Actuator command limits/1 -> [limited_command], command/1
  Integral action/1 -> [integral_command]
  PI plus holding command/1 -> Actuator command limits/1, [raw_command]
  Integral input/1 -> Integral action/1
  Holding command/1 -> PI plus holding command/3
  error_N/1 -> estimated_force_error_N/1, Force controller sampling/1
  measured_travel_m/1 -> estimated_travel_m/1
  [force_error_N] -> Integral gain/1
  [force_error_N] -> Filtered force derivative/1
  Derivative gain/1 -> [derivative_command]
  Saturation error/1 -> Anti windup/1
  [limited_command] -> Saturation error/1
  Force controller sampling/1 -> Proportional gain/1, [force_error_N]
  Anti windup/1 -> [tracking_correction]
  [raw_command] -> Saturation error/2
  Integral gain/1 -> Integral input/1
  [derivative_command] -> PI plus holding command/4
  [integral_command] -> PI plus holding command/2
  Filtered force derivative/1 -> Derivative gain/1
  [tracking_correction] -> Integral input/2
  Proportional gain/1 -> PI plus holding command/1

== system acf_rl_native/Force measurement/Engineered common AA and EMA ==
  analog input : Inport
  ADC analog input filter : StateSpace  A=p.adcStudy.d.converterAnalog.A  B=p.adcStudy.d.converterAnalog.B  C=p.adcStudy.d.converterAnalog.C  D=p.adcStudy.d.converterAnalog.D  InitialCondition=((p.force.reference*(1+p.uncertainty.forceScaleZ)*(cos(p.uncertainty.forceFrameAngle_rad)-p.contact.mu*(sin(p.uncertainty.forceFrameAngle_rad)+p.uncertainty.forceCrossZFromX))))*p.adcStudy.d.converterAnalog.steadyStatePerUnitInput
  ADC clipping magnitude : Abs  SaturateOnIntegerOverflow=off
  ADC input and output noise : Sum
  ADC output noise correlation : DiscreteTransferFcn  Numerator=p.adcStudy.d.converterNoise.numerator  Denominator=p.adcStudy.d.converterNoise.denominator  SampleTime=p.adcStudy.outputSampleTime_s
  ADC range difference : Sum  Inputs=+-
  Actual ADC input range : Saturate  UpperLimit=p.adcStudy.forceAdcRange_N  LowerLimit=-(p.adcStudy.forceAdcRange_N)
  Actual ADC output samples : ZeroOrderHold  SampleTime=p.adcStudy.outputSampleTime_s
  Actual converter quantization : Quantizer  QuantizationInterval=max(p.adcStudy.forceQuantum_N,1e-15)
  Continuous analog front end : StateSpace  A=p.adcStudy.d.channels.force.analogA  B=p.adcStudy.d.channels.force.analogB  C=p.adcStudy.d.channels.force.analogC  D=p.adcStudy.d.channels.force.analogD  InitialCondition=((p.force.reference*(1+p.uncertainty.forceScaleZ)*(cos(p.uncertainty.forceFrameAngle_rad)-p.contact.mu*(sin(p.uncertainty.forceFrameAngle_rad)+p.uncertainty.forceCrossZFromX))))*p.adcStudy.d.channels.force.analogSteadyStatePerUnitInput
  Converter output noise RMS : Gain  Gain=p.adcStudy.forceAdcNoiseRms_N
  Fresh per-conversion EMA : DiscreteTransferFcn  Numerator=p.adcStudy.d.channels.force.emaNumerator  Denominator=p.adcStudy.d.channels.force.emaDenominator  InitialStates=(round((((p.force.reference*(1+p.uncertainty.forceScaleZ)*(cos(p.uncertainty.forceFrameAngle_rad)-p.contact.mu*(sin(p.uncertainty.forceFrameAngle_rad)+p.uncertainty.forceCrossZFromX))))+(p.adcStudy.d.forceGravityOffset_N))/(max(p.adcStudy.forceQuantum_N,1e-15)))*(max(p.adcStudy.forceQuantum_N,1e-15))-round((p.adcStudy.d.forceGravityOffset_N)/(max(p.adcStudy.forceQuantum_N,1e-15)))*(max(p.adcStudy.forceQuantum_N,1e-15)))*p.adcStudy.d.channels.force.emaSteadyStatePerUnitInput  SampleTime=p.adcStudy.outputSampleTime_s
  Independent converter output noise : RandomNumber  Seed=p.sensor.seed+2594  SampleTime=p.adcStudy.outputSampleTime_s
  Known quantized static offset : Bias  Bias=-round((p.adcStudy.d.forceGravityOffset_N)/(max(p.adcStudy.forceQuantum_N,1e-15)))*(max(p.adcStudy.forceQuantum_N,1e-15))  SaturateOnIntegerOverflow=off
  Native converter impulse response : DiscreteTransferFcn  Numerator=p.adcStudy.d.converter.numerator  Denominator=p.adcStudy.d.converter.denominator  InitialStates=((p.force.reference*(1+p.uncertainty.forceScaleZ)*(cos(p.uncertainty.forceFrameAngle_rad)-p.contact.mu*(sin(p.uncertainty.forceFrameAngle_rad)+p.uncertainty.forceCrossZFromX))))*p.adcStudy.d.converter.steadyStatePerUnitInput  SampleTime=p.adcStudy.fineClock_s
  Restore physical static offset : Bias  Bias=p.adcStudy.d.forceGravityOffset_N  SaturateOnIntegerOverflow=off
  conditioned output : Outport
  tag scope: force_adc_clip=global, force_adc_prequant=global
  wires:
  Actual ADC output samples/1 -> ADC input and output noise/1
  Independent converter output noise/1 -> Converter output noise RMS/1
  Converter output noise RMS/1 -> ADC output noise correlation/1
  ADC output noise correlation/1 -> ADC input and output noise/2
  ADC input and output noise/1 -> Restore physical static offset/1
  Restore physical static offset/1 -> Actual ADC input range/1, [force_adc_prequant], ADC range difference/1
  Actual ADC input range/1 -> Actual converter quantization/1, ADC range difference/2
  Actual converter quantization/1 -> Known quantized static offset/1
  ADC range difference/1 -> ADC clipping magnitude/1
  ADC clipping magnitude/1 -> [force_adc_clip]
  analog input/1 -> Continuous analog front end/1
  Continuous analog front end/1 -> ADC analog input filter/1
  ADC analog input filter/1 -> Native converter impulse response/1
  Native converter impulse response/1 -> Actual ADC output samples/1
  Known quantized static offset/1 -> Fresh per-conversion EMA/1
  Fresh per-conversion EMA/1 -> conditioned output/1

== system acf_rl_native/Lateral B-S force measurement/Engineered common AA and EMA ==
  analog input : Inport
  ADC analog input filter : StateSpace  A=p.adcStudy.d.converterAnalog.A  B=p.adcStudy.d.converterAnalog.B  C=p.adcStudy.d.converterAnalog.C  D=p.adcStudy.d.converterAnalog.D  InitialCondition=((p.force.reference*(1+p.uncertainty.forceScaleX)*(-p.contact.mu*cos(p.uncertainty.forceFrameAngle_rad)-sin(p.uncertainty.forceFrameAngle_rad)+p.uncertainty.forceCrossXFromZ)))*p.adcStudy.d.converterAnalog.steadyStatePerUnitInput
  ADC clipping magnitude : Abs  SaturateOnIntegerOverflow=off
  ADC input and output noise : Sum
  ADC output noise correlation : DiscreteTransferFcn  Numerator=p.adcStudy.d.converterNoise.numerator  Denominator=p.adcStudy.d.converterNoise.denominator  SampleTime=p.adcStudy.outputSampleTime_s
  ADC range difference : Sum  Inputs=+-
  Actual ADC input range : Saturate  UpperLimit=p.adcStudy.forceAdcRange_N  LowerLimit=-(p.adcStudy.forceAdcRange_N)
  Actual ADC output samples : ZeroOrderHold  SampleTime=p.adcStudy.outputSampleTime_s
  Actual converter quantization : Quantizer  QuantizationInterval=max(p.adcStudy.forceQuantum_N,1e-15)
  Continuous analog front end : StateSpace  A=p.adcStudy.d.channels.lateral.analogA  B=p.adcStudy.d.channels.lateral.analogB  C=p.adcStudy.d.channels.lateral.analogC  D=p.adcStudy.d.channels.lateral.analogD  InitialCondition=((p.force.reference*(1+p.uncertainty.forceScaleX)*(-p.contact.mu*cos(p.uncertainty.forceFrameAngle_rad)-sin(p.uncertainty.forceFrameAngle_rad)+p.uncertainty.forceCrossXFromZ)))*p.adcStudy.d.channels.lateral.analogSteadyStatePerUnitInput
  Converter output noise RMS : Gain  Gain=p.adcStudy.forceAdcNoiseRms_N
  Fresh per-conversion EMA : DiscreteTransferFcn  Numerator=p.adcStudy.d.channels.lateral.emaNumerator  Denominator=p.adcStudy.d.channels.lateral.emaDenominator  InitialStates=(round((((p.force.reference*(1+p.uncertainty.forceScaleX)*(-p.contact.mu*cos(p.uncertainty.forceFrameAngle_rad)-sin(p.uncertainty.forceFrameAngle_rad)+p.uncertainty.forceCrossXFromZ)))+(p.adcStudy.d.lateralGravityOffset_N))/(max(p.adcStudy.forceQuantum_N,1e-15)))*(max(p.adcStudy.forceQuantum_N,1e-15))-round((p.adcStudy.d.lateralGravityOffset_N)/(max(p.adcStudy.forceQuantum_N,1e-15)))*(max(p.adcStudy.forceQuantum_N,1e-15)))*p.adcStudy.d.channels.lateral.emaSteadyStatePerUnitInput  SampleTime=p.adcStudy.outputSampleTime_s
  Independent converter output noise : RandomNumber  Seed=p.sensor.seed+2808  SampleTime=p.adcStudy.outputSampleTime_s
  Known quantized static offset : Bias  Bias=-round((p.adcStudy.d.lateralGravityOffset_N)/(max(p.adcStudy.forceQuantum_N,1e-15)))*(max(p.adcStudy.forceQuantum_N,1e-15))  SaturateOnIntegerOverflow=off
  Native converter impulse response : DiscreteTransferFcn  Numerator=p.adcStudy.d.converter.numerator  Denominator=p.adcStudy.d.converter.denominator  InitialStates=((p.force.reference*(1+p.uncertainty.forceScaleX)*(-p.contact.mu*cos(p.uncertainty.forceFrameAngle_rad)-sin(p.uncertainty.forceFrameAngle_rad)+p.uncertainty.forceCrossXFromZ)))*p.adcStudy.d.converter.steadyStatePerUnitInput  SampleTime=p.adcStudy.fineClock_s
  Restore physical static offset : Bias  Bias=p.adcStudy.d.lateralGravityOffset_N  SaturateOnIntegerOverflow=off
  conditioned output : Outport
  tag scope: lateral_adc_clip=global, lateral_adc_prequant=global
  wires:
  Actual ADC output samples/1 -> ADC input and output noise/1
  Independent converter output noise/1 -> Converter output noise RMS/1
  Converter output noise RMS/1 -> ADC output noise correlation/1
  ADC output noise correlation/1 -> ADC input and output noise/2
  ADC input and output noise/1 -> Restore physical static offset/1
  Restore physical static offset/1 -> Actual ADC input range/1, [lateral_adc_prequant], ADC range difference/1
  Actual ADC input range/1 -> Actual converter quantization/1, ADC range difference/2
  Actual converter quantization/1 -> Known quantized static offset/1
  ADC range difference/1 -> ADC clipping magnitude/1
  ADC clipping magnitude/1 -> [lateral_adc_clip]
  analog input/1 -> Continuous analog front end/1
  Continuous analog front end/1 -> ADC analog input filter/1
  ADC analog input filter/1 -> Native converter impulse response/1
  Native converter impulse response/1 -> Actual ADC output samples/1
  Known quantized static offset/1 -> Fresh per-conversion EMA/1
  Fresh per-conversion EMA/1 -> conditioned output/1
